simulink model "EncoderToRPM"  (R2026b)
settings: Solver=VariableStepAuto
values from neighbouring files (symbols this model uses):
  Enc_RPMGain = Enc_Dir*Enc_Kcal*60/(Ts*Enc_CountsPerRev)    (= 23.5340909091)    [DCMotorParams.m]
  RPM_LPF_Den = [1, RPM_LPF_a - 1]    [DCMotorParams.m]
  RPM_LPF_Num = RPM_LPF_a    (= 0.2)    [DCMotorParams.m]
  Ts = 0.01    [DCMotorParams.m]
libraries: simulink x1, arduinosensorlib x1
settings Model: Creator=bence  LastModifiedBy=bence

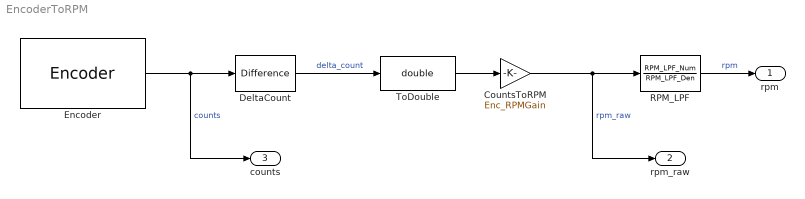
== system EncoderToRPM ==
  CountsToRPM : Gain  Gain=Enc_RPMGain
  DeltaCount : simulink/Discrete/Difference  ICPrevInput=0  OutMin=[]  OutMax=[]  OutDataTypeStr=int32  OutputDataTypeScalingMode=int32  OutDataType=fixdt(1, 16)  OutScaling=2^-10  DoSatur=off
  Encoder : arduinosensorlib/Encoder  InputA=2  InputB=3  Mode=No reset  SampleTime=Ts
  RPM_LPF : DiscreteTransferFcn  Numerator=RPM_LPF_Num  Denominator=RPM_LPF_Den  SampleTime=Ts
  ToDouble : DataTypeConversion  OutDataTypeStr=double  SaturateOnIntegerOverflow=off  RndMeth=Floor
  rpm : Outport
  rpm_raw : Outport  Port=2
  counts : Outport  Port=3
  wires:
  DeltaCount/1 -> ToDouble/1  "delta_count"
  ToDouble/1 -> CountsToRPM/1
  CountsToRPM/1 -> rpm_raw/1, RPM_LPF/1  "rpm_raw"
  RPM_LPF/1 -> rpm/1  "rpm"
  Encoder/1 -> counts/1, DeltaCount/1  "counts"
